simulink model "BalancingRobot"  (Simulink 7.1)
settings: Solver=ode5  StartTime=0.0  StopTime=1  FixedStep=.02  RelTol=1e-3
undefined symbols (not defined in the file or in its folder): Az, Bz, Cz, Dz, K
settings Model: Creator=gauss  LastModifiedBy=Lubin
settings DebuggingCC: SignalResolutionControl=TryResolveAllWithWarning  MultiTaskDSMMsg=warning  MultiTaskCondExecSysMsg=none
settings HardwareCC: TargetHWDeviceType=32-bit Generic
settings GRTTargetCC: TargetFcnLib=ansi_tfl_tmw.mat

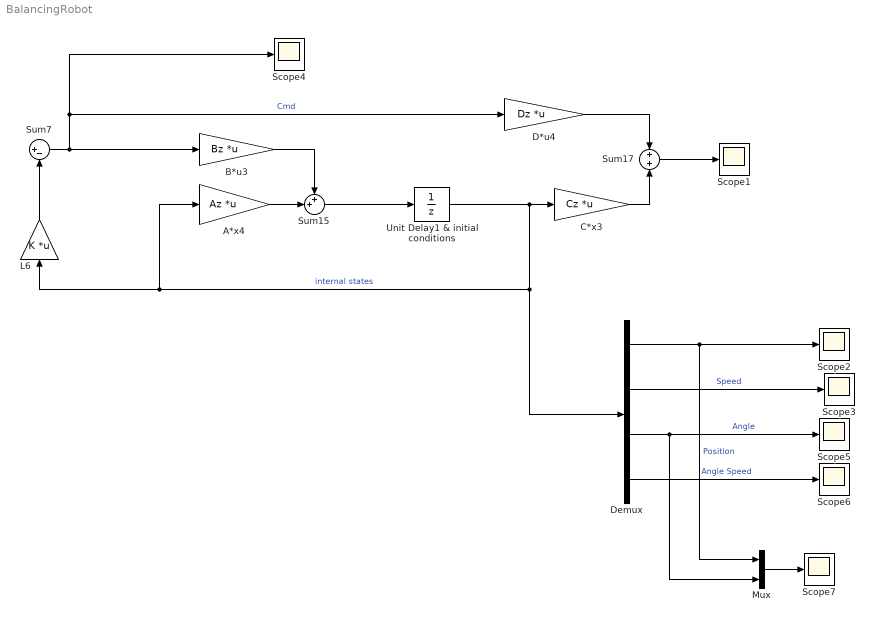
== system BalancingRobot ==
  A*x4 : Gain  Gain=Az  Multiplication=Matrix(K*u) (u vector)  ParameterDataType=sfix(16)  ParameterScaling=2^0  OutDataTypeMode=double  OutDataType=fixdt(1,32,16)  OutDataTypeStr=double  SaturateOnIntegerOverflow=on
  B*u3 : Gain  Gain=Bz  Multiplication=Matrix(K*u) (u vector)  ParameterDataType=sfix(16)  ParameterScaling=2^0  OutDataTypeMode=double  OutDataType=fixdt(1,32,20)  OutDataTypeStr=double  SaturateOnIntegerOverflow=on
  C*x3 : Gain  Gain=Cz  Multiplication=Matrix(K*u) (u vector)  ParameterDataType=sfix(16)  ParameterScaling=2^0  OutDataTypeMode=double  OutDataType=fixdt(1,32,20)  OutDataTypeStr=double
  D*u4 : Gain  Gain=Dz  Multiplication=Matrix(K*u) (u vector)  ParameterDataType=sfix(16)  ParameterScaling=2^0  OutDataTypeMode=double  OutDataType=fixdt(1,32,26)  OutDataTypeStr=double  SaturateOnIntegerOverflow=on
  Demux : Demux
  L6 : Gain  Orientation=up  Gain=K  Multiplication=Matrix(K*u) (u vector)  ParameterDataType=sfix(16)  ParameterScaling=2^0  OutDataTypeMode=double  OutDataType=fixdt(1,32,18)  OutDataTypeStr=double
  Mux : Mux  Inputs=2
  Scope{1..7} (7 alike) : Scope
      Scope1 settings: TimeRange=0.2  YMin=-10000  YMax=5000
      Scope2 settings: TimeRange=0.2  YMin=-10000  YMax=5000
      Scope3 settings: TimeRange=0.2  YMin=-10000  YMax=5000  SaveName=ScopeData2
      Scope4 settings: TimeRange=0.2  YMin=-10000  YMax=5000  SaveName=ScopeData3
      Scope5 settings: TimeRange=0.2  YMin=-10000  YMax=5000  SaveName=ScopeData4
      Scope6 settings: TimeRange=0.2  YMin=-10000  YMax=5000  SaveName=ScopeData5
      Scope7 settings: TimeRange=0.2  YMin=-10000  YMax=5000  SaveName=ScopeData6
  Sum15 : Sum  Inputs=++|  OutDataTypeMode=double  OutDataType=fixdt(1,32,17)  OutDataTypeStr=double
  Sum17 : Sum  OutDataTypeMode=double  OutDataType=fixdt(1,32,23)  OutDataTypeStr=double  SaturateOnIntegerOverflow=on
  Sum7 : Sum  Inputs=|+-  OutDataTypeMode=double  OutDataType=fixdt(1,32,19)  OutDataTypeStr=double  SaturateOnIntegerOverflow=on
  Unit Delay1 & initial conditions : UnitDelay  X0=[.1 0 0 0]  SampleTime=-1
  wires:
  L6/1 -> Sum7/2
  Unit Delay1 & initial conditions/1 -> C*x3/1, L6/1, A*x4/1, Demux/1  "internal states"
  Sum7/1 -> B*u3/1, D*u4/1, Scope4/1  "Cmd"
  A*x4/1 -> Sum15/2
  B*u3/1 -> Sum15/1
  Sum15/1 -> Unit Delay1 & initial conditions/1
  C*x3/1 -> Sum17/2
  D*u4/1 -> Sum17/1
  Sum17/1 -> Scope1/1
  Demux/1 -> Scope2/1, Mux/1  "Position"
  Demux/2 -> Scope3/1  "Speed"
  Demux/3 -> Scope5/1, Mux/2  "Angle"
  Demux/4 -> Scope6/1  "Angle Speed"
  Mux/1 -> Scope7/1
